simulink model "Lab2_VM_Task_1234"  (R2026a)
settings: Solver=FixedStepDiscrete  StopTime=inf  FixedStep=0.02  EnableMultiTasking=on
undefined symbols (not defined in the file or in its folder): Angular, Linear
libraries: robotlib x3
settings Model: Creator=The MathWorks, Inc.  LastModifiedBy=juulg
settings OptimizationCC: LifeSpan=Inf
settings HardwareCC: ProdHWDeviceType=Generic->Unspecified (assume 32-bit Generic)  TargetHWDeviceType=Generic->Unspecified (assume 32-bit Generic)  UseEmbeddedCoderFeatures=off
settings SFSimCC: SimTargetLang=C++
settings RTWCC: SystemTargetFile=ert.tlc  HardwareBoard=Robot Operating System (ROS)  Toolchain=Catkin  TargetLang=C++  Description=Embedded Coder
settings ERTTargetCC: RootIOFormat=Structure reference  DynamicArrayContainerType=coder::array  MultiwordLength=2048.0  ERTCustomFileBanners=off  CodeInterfacePackaging=C++ class  SubcomponentCodeInterfacePackaging=C++ class  SupportContinuousTime=on  SupportNonInlinedSFcns=on  SupportVariableSizeSignals=on  ModelStepFunctionPrototypeControlCompliant=off

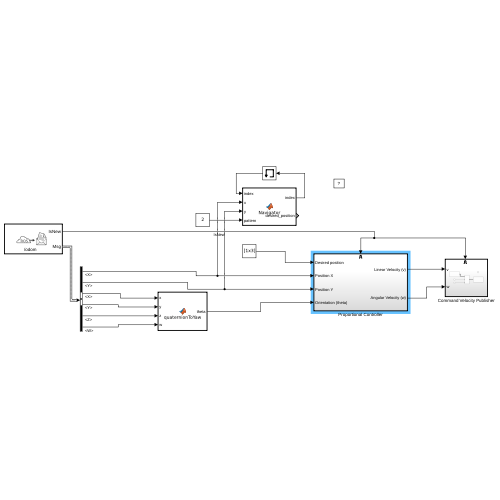
[thumbnail: Simulink's stored preview of the top-level diagram]
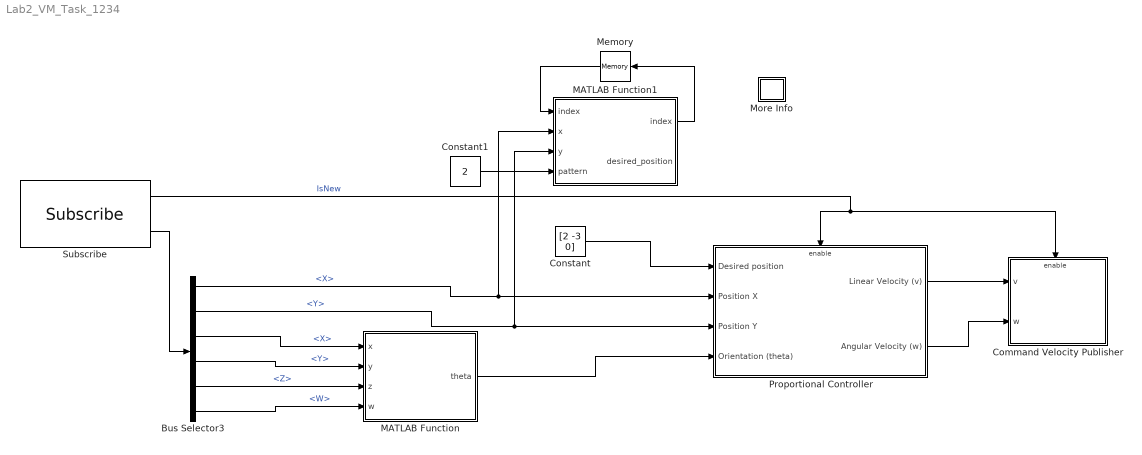
== system Lab2_VM_Task_1234 ==
  Bus Selector3 : BusSelector  OutputSignals=Pose.Pose.Position.X,Pose.Pose.Position.Y,Pose.Pose.Orientation.X,Pose.Pose.Orientation.Y,Pose.Pose.Orientation.Z,Pose.Pose.Orientation.W
  Command Velocity Publisher : Subsystem
  Constant : Constant  Value=[2 -3 0]  VectorParams1D=off
  Constant1 : Constant  Value=2
  MATLAB Function : MATLAB Function  TreatAsAtomicUnit=on
  MATLAB Function1 : MATLAB Function  TreatAsAtomicUnit=on
  Memory : Memory  InitialCondition=1
  More Info : Subsystem
      settings: OpenFcn=showdemo(bdroot(gcb))
      mask Display: disp('?')
  Proportional Controller : Subsystem
  Subscribe : robotlib/Subscribe  topicSource=Select from ROS network  topic=/odom  messageType=nav_msgs/Odometry  SampleTime=-1  legacyBusStruct=off  messageQueueLength=51
  wires:
  Subscribe/2 -> Bus Selector3/1
  Proportional Controller/1(Linear Velocity (v)) -> Command Velocity Publisher/1(v)
  Subscribe/1 -> Command Velocity Publisher/Enable, Proportional Controller/Enable  "IsNew"
  Bus Selector3/4 -> MATLAB Function/2(y)  "<Y>"
  Proportional Controller/2(Angular Velocity (w)) -> Command Velocity Publisher/2(w)
  Bus Selector3/2 -> MATLAB Function1/3(y), Proportional Controller/3(Position Y)  "<Y>"
  Bus Selector3/1 -> MATLAB Function1/2(x), Proportional Controller/2(Position X)  "<X>"
  MATLAB Function/1(theta) -> Proportional Controller/4(Orientation (theta))
  Bus Selector3/6 -> MATLAB Function/4(w)  "<W>"
  Bus Selector3/5 -> MATLAB Function/3(z)  "<Z>"
  Bus Selector3/3 -> MATLAB Function/1(x)  "<X>"
  MATLAB Function1/1(index) -> Memory/1
  Memory/1 -> MATLAB Function1/1("index ")
  Constant1/1 -> MATLAB Function1/4(pattern)
  Constant/1 -> Proportional Controller/1(Desired position)

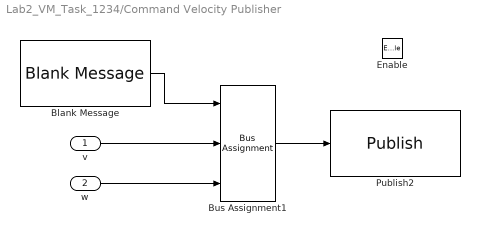
== system Lab2_VM_Task_1234/Command Velocity Publisher ==
  v : Inport
  w : Inport  Port=2
  Enable : EnablePort
  Blank Message : robotlib/Blank Message  messageClass=Message  entityType=geometry_msgs/Twist  messageType=geometry_msgs/Twist  SampleTime=inf  legacyBusStruct=off
  Bus Assignment1 : BusAssignment  DialogController=Simulink.DDGSource_BusAssignment  AssignedSignals=Linear.X,Angular.Z
  Publish2 : robotlib/Publish  topicSource=Select from ROS network  topic=/cmd_vel  messageType=geometry_msgs/Twist  legacyBusStruct=off  messageQueueLength=105
  wires:
  Bus Assignment1/1 -> Publish2/1
  Blank Message/1 -> Bus Assignment1/1
  v/1 -> Bus Assignment1/2
  w/1 -> Bus Assignment1/3

== system Lab2_VM_Task_1234/More Info ==

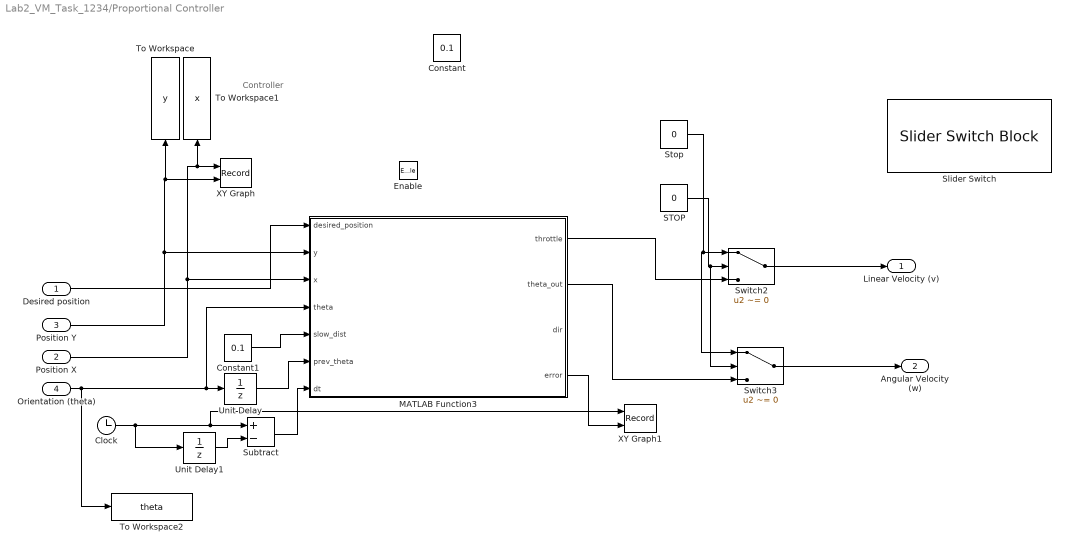
== system Lab2_VM_Task_1234/Proportional Controller ==
  note: Controller
  Desired position : Inport
  Position X : Inport  Port=2
  Position Y : Inport  Port=3
  Orientation (theta) : Inport  Port=4
  Enable : EnablePort
  Clock : Clock
  Constant : Constant  Value=0.1
  Constant1 : Constant  Value=0.1
  MATLAB Function3 : MATLAB Function  TreatAsAtomicUnit=on
  "STOP " : Constant  Value=0
  Slider Switch : SliderSwitchBlock
  Stop : Constant  Value=0
  Subtract : Sum  Inputs=+-
  Switch2 : Switch  Criteria=u2 ~= 0  SaturateOnIntegerOverflow=off  InputSameDT=off
  Switch3 : Switch  Criteria=u2 ~= 0  SaturateOnIntegerOverflow=off  InputSameDT=off
  To Workspace : ToWorkspace  VariableName=y  SaveFormat=Timeseries  SampleTime=-1
  To Workspace1 : ToWorkspace  VariableName=x  SaveFormat=Timeseries  SampleTime=-1
  To Workspace2 : ToWorkspace  VariableName=theta  SaveFormat=Timeseries  SampleTime=-1
  Unit Delay : UnitDelay  SampleTime=-1
  Unit Delay1 : UnitDelay  SampleTime=-1
  XY Graph : Record  NumPorts=2.0  FileSettingsInternal="{\"entries\":[{\"content\":{\"excelSettings\":{\"content\":{},\"type\":\"Streamout.ExcelSettings\"},\"parquetSettings\":{\"content\":{},\"type\":\"Streamout.ParquetSettings\"}},\"type\":\"Streamout.FileSettingStorage\",\"uuid\":\"\"}],\"packageUris\":[\"http:\\/\\/schema.mathworks.com\\/mf0\\/streamout_blocks\\/R2020a\"],\"version\":\"1.0\"}"  FrameSettings=[0, 0]  Layout=[1 1]  SignalsInternal="{\"entries\":[{\"content\":{\"signals\":[{\"content\":{\"blockPath\":[],\"dimensions\":[1],\"domain\":\"\",\"lineColor\":\"#a2142f\",\"plots\":[ 1 ],\"port\":1,\"sid\":[\"\"],\"signalID\":1,\"signalName\":\"X\"},\"type\":\"RecordBlkView.Signal\",\"uuid\":\"\"},{\"content\":{\"blockPath\":[],\"dimensions\":[1],\"domain\":\"\",\"lineColor\":\"#139fff\",\"plots\":[ 1 ],\"port\":2,\"sid\":[\"\"],\"signalID\":2,\"signalName\":\"Y\"},\"type\":\"RecordBlkView.Signal\",\"uuid\":\"\"}]},\"type\":\"RecordBlkView.InputSignals\",\"uuid\":\"\"}],\"packageUris\":[\"http:\\/\\/schema.mathworks.com\\/mf0\\/streamout_blocks\\/R2020a\"],\"version\":\"1.0\"}"  VisualizationBindings="{\"xyplotplugin\":{\"info\":[{\"series\":[{\"bindingParametersList\":[{\"parameter\":\"X-Axis\",\"signalID\":1,\"signalName\":\"X\"},{\"parameter\":\"Y-Axis\",\"signalID\":2,\"signalName\":\"Y\"}],\"seriesID\":0}],\"subplotID\":1}]}}"  CompatibilityTag=XY
  XY Graph1 : Record  NumPorts=2.0  FileSettingsInternal="{\"entries\":[{\"content\":{\"excelSettings\":{\"content\":{},\"type\":\"Streamout.ExcelSettings\"},\"parquetSettings\":{\"content\":{},\"type\":\"Streamout.ParquetSettings\"}},\"type\":\"Streamout.FileSettingStorage\",\"uuid\":\"\"}],\"packageUris\":[\"http:\\/\\/schema.mathworks.com\\/mf0\\/streamout_blocks\\/R2020a\"],\"version\":\"1.0\"}"  FrameSettings=[0, 0]  Layout=[1 1]  SignalsInternal="{\"entries\":[{\"content\":{\"signals\":[{\"content\":{\"blockPath\":[],\"dimensions\":[1],\"domain\":\"\",\"lineColor\":\"#a2142f\",\"plots\":[ 1 ],\"port\":1,\"sid\":[\"\"],\"signalID\":1,\"signalName\":\"Clock\"},\"type\":\"RecordBlkView.Signal\",\"uuid\":\"\"},{\"content\":{\"blockPath\":[],\"dimensions\":[1],\"domain\":\"\",\"lineColor\":\"#139fff\",\"plots\":[ 1 ],\"port\":2,\"sid\":[\"\"],\"signalID\":2,\"signalName\":\"MATLAB Function3:4\"},\"type\":\"RecordBlkView.Signal\",\"uuid\":\"\"}]},\"type\":\"RecordBlkView.InputSignals\",\"uuid\":\"\"}],\"packageUris\":[\"http:\\/\\/schema.mathworks.com\\/mf0\\/streamout_blocks\\/R2020a\"],\"version\":\"1.0\"}"  VisualizationBindings="{\"xyplotplugin\":{\"info\":[{\"series\":[{\"bindingParametersList\":[{\"parameter\":\"X-Axis\",\"signalID\":1,\"signalName\":\"Clock\"},{\"parameter\":\"Y-Axis\",\"signalID\":2,\"signalName\":\"MATLAB Function3:4\"}],\"seriesID\":0}],\"subplotID\":1}]}}"  CompatibilityTag=XY
  Linear Velocity (v) : Outport  VectorParamsAs1DForOutWhenUnconnected=off
  Angular Velocity (w) : Outport  Port=2  VectorParamsAs1DForOutWhenUnconnected=off
  wires:
  Stop/1 -> Switch3/1, Switch2/1
  "STOP "/1 -> Switch3/2, Switch2/2
  Switch2/1 -> Linear Velocity (v)/1
  Switch3/1 -> Angular Velocity (w)/1
  Orientation (theta)/1 -> Unit Delay/1, MATLAB Function3/4(theta), To Workspace2/1
  Position X/1 -> To Workspace1/1, XY Graph/1, MATLAB Function3/3(x)
  Position Y/1 -> To Workspace/1, XY Graph/2, MATLAB Function3/2(y)
  Desired position/1 -> MATLAB Function3/1(desired_position)
  Constant1/1 -> MATLAB Function3/5(slow_dist)
  MATLAB Function3/1(throttle) -> Switch2/3
  MATLAB Function3/2(theta_out) -> Switch3/3
  Unit Delay/1 -> MATLAB Function3/6(prev_theta)
  Clock/1 -> Unit Delay1/1, XY Graph1/1, Subtract/1
  Unit Delay1/1 -> Subtract/2
  Subtract/1 -> MATLAB Function3/7(dt)
  MATLAB Function3/4(error) -> XY Graph1/2

== matlab function Lab2_VM_Task_1234/MATLAB Function1 ==
  data: index output; index input; desired_position output; x input; y input; pattern input
function [index,desired_position] = Navigator(index, x,y, pattern)
    square_motion = [0 10; 10 10; 10 0; 0 0];
    j_motion = [
    0 0;
    5.6533 0;
    5.6533 -8.1659;
    3.3501 -9.4221;
    0.8375 -9.2128;
    0 -7.3283
    ];
    i = linspace(0,360,20).';
    sin_motion = [i/9, 10*sin(deg2rad(i))];
    straight_motion=[i,zeros(1, length(i))'];
    % Store paths in a cell array
    patterns = {square_motion, j_motion, sin_motion, straight_motion};

    % Select current path
    current_pattern = patterns{pattern};

    % Get current waypoint
    desired_position = current_pattern(index,:);

    % Check distance to waypoint
    if norm(desired_position(1:2) - [x y]) < 0.12

        index = mod(index, size(current_pattern,1)) + 1;

        % Update desired waypoint
        desired_position = current_pattern(index,:);
    end
end

== matlab function Lab2_VM_Task_1234/MATLAB Function ==
  data: x input; theta output; y input; z input; w input
function theta = quaternionToYaw(x,y,z,w)

    theta = atan2(2*(w*z + x*y), ...
                  1 - 2*(y*y + z*z));

end

== matlab function Lab2_VM_Task_1234/Proportional Controller/MATLAB Function3 ==
  data: throttle output; desired_position input; theta_out output; y input; x input; theta input; slow_dist input; dir output; prev_theta input; dt input; error output
function [throttle, theta_out, dir, error] = controller(desired_position,y,x,theta, slow_dist, prev_theta, dt)
    slow_speed=0.01;
    d_theta =-1;
    if (length(desired_position)>2)
        d_theta = desired_position(3);
        %desired_position = desired_position(1:2);
    end
    position = [x y];
    Kp = 0.2;
    Kd= 0.2;
    %x2=desired_position[1];
    %y2=desired_position[2];
    
    % Get direction towards goal
    direction =desired_position(1:2)-position;
    distance= norm(direction);
    dir = atan2(direction(2),direction(1));
    theta_diff = mod(theta-prev_theta + pi, 2*pi) - pi;
    if distance < slow_dist
        if (d_theta==-1)
            theta_out = 0;
            throttle = 0;
            error=0;
            return;
        end            
        % Final orientation error
        error = mod(d_theta - theta + pi, 2*pi) - pi;

        % Angular velocity
        theta_rate = theta_diff / dt;

        % Controller gains
        Kp_final = 0.8;
        Kd_final = 0.3;

        % PD controller
        theta_out = Kp_final*error - Kd_final*theta_rate;

        % Limit angular velocity
        max_angular = 0.3;
        theta_out = max(min(theta_out, max_angular), -max_angular);

        % Stopping condition
        if abs(error) < 0.03 && abs(theta_rate) < 0.04
            theta_out = 0;
            throttle = 0;
            return;
        end

        % Low forward velocity during final alignment
        %throttle = slow_speed;
        throttle=0;
        return;
    end
    error = mod(dir-theta + pi, 2*pi) - pi;
    % Compare with current heading
    
    % Deciding direction to rotate
    theta_out=error*Kp- (theta_diff/(dt+1e-5))*Kd;
    theta_out=clip(theta_out,-0.5,0.5);
    %throttle = 0.5 * max(0, 1 - abs(error)/pi);
    if(abs(error)>0.05)
        %throttle = slow_speed;
        throttle=0;
    else
        %throttle = 0.5*cos(error*15);
        throttle = 0.1;
    end
end
